simulink model "DATCOM_SimulinkModel"  (R2026a)
settings: Solver=ode4  StopTime=120  FixedStep=params.DT
InitFcn:
  | % Place this in SITL_SimulinkModel > Model Properties > Call Backs >
  | % InitFcn to initialize the states and stuff
  | fprintf("~~~~ Ardupilot SITL Time ~~~~~");
  | clear SITL_Link_Step
  | clear SITL_Bridge_Step
  | 
  | params = SITL_RascalParams();
  | paramsD = DATCOM_RascalParams();
  | params.DT = 1/1200;
  | 
  | %% Initial attitude
  | % Enter the required euler angles here
  | p = deg2rad(0);   % Phi - Roll angle
  | t = deg2rad(0);   % Theta - Pitch angle
  | s = deg2rad(0);   % Psi - Yaw angle
  | q = eul2quat([s t p]);
  | 
  | %% Initial velocity
  | % Glide test: 16 m/s along body x only, so AoA = 0
  | % (for level flight at a pitch angle use u = V*cos(t), w = V*sin(t))
  | u = 40;
  | w = 0;
  | 
  | %% Initial state
  | % Runway start (taildragger rest attitude)
  | % theta0 = deg2rad(14.3);
  | % X0 = [0;0;-0.4;  0;0;0;   cos(theta0/2);0;sin(theta0/2);0;  0;0;0];
  | X0 = [0;0;-2000;  16;0;0;  q';  0;0;0];    % 2000 m up so it doesn't hit the ground, north
  | 
  | %% Actuators and prop
  | PWM0 = 1500*ones(16,1);   % This is the systematic delay or else
  | % simulink thinks everything is happening at once!
  | delta0 = [0;0;0;0];       % For the aileron, elevator, rudder and throttle
  | % We are not considering a special one for the throttle as well
  | % This should also become the trim states if you are trying to
  | % start the SITL from a point in the Air
  | omega0 = 0;
  | 
  | %% Test PWM (throttle off). Elevator PWM sets the glide speed, 1500 = 0 rad
  | % above 1500 = nose up: dE = -(PWM-1500)/400*0.35 rad, e.g. 1569 -> -0.06
  | PWM_TEST = 1500*ones(16,1);
  | PWM_TEST(2) = 1580;
  | PWM_TEST(3) = 1100;
  | 
  | fprintf("~~~~ INITIALIZED ~~~~~");
StopFcn:
  | clear SITL_Link_Step
  | clear SITL_Bridge_Step
libraries: simulink_extras x3
settings Model: SimulationMode=accelerator  Creator=kiryuzerodev  LastModifiedBy=kiryuzerodev

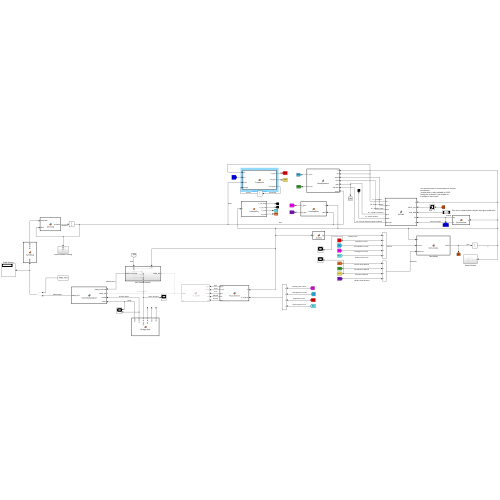
[thumbnail: Simulink's stored preview of the top-level diagram]
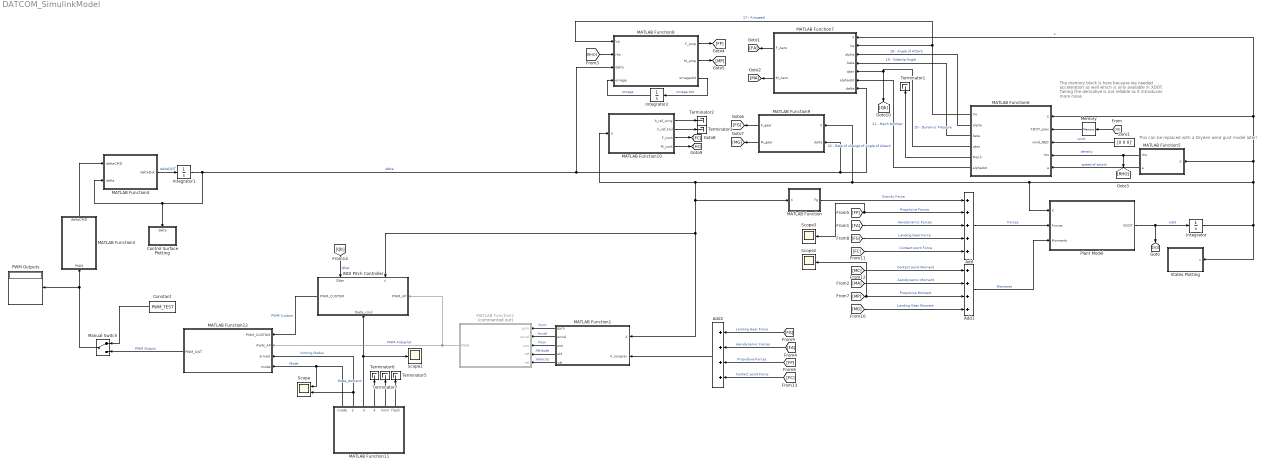
== system DATCOM_SimulinkModel ==
  note: The memory block is here because we needed acceleration
      |  as well which is only available in XDOT.
      | Taking the derivative is not reliable as
      | it introduces more noise
  note: This can be replaced with a Dryden wind gust model later!
  Add : Sum  Inputs=+++++
  Add1 : Sum  Inputs=++++
  Add2 : Sum  Inputs=++++
  Constant : Constant  Value=PWM_TEST
  Control Surface Plotting : Subsystem
  INDI Pitch Controller : Subsystem  TreatAsAtomicUnit=on
      settings: PortSchema="{\"entries\":[{\"content\":{\"sides\":[{\"content\":{\"connectorIds\":[\"In1\"]},\"type\":\"ConnectorPlacement.EquallySpacedRectSide\",\"uuid\":\"6d37aedf-8600-4591-b995-97b477a77a55\"},{\"content\":{\"connectorIds\":[\"Out1\"],\"side\":\"RIGHT\"},\"type\":\"ConnectorPlacement.EquallySpacedRectSide\",\"uuid\":\"78620349-e441-4417-9f68-6134c6dddec3\"},{\"content\":{\"connectorIds\":[\"In2\",\"In3\"],\"side\":\"TOP\"},\"type\":\"ConnectorPlacement.EquallySpacedRectSide\",\"uuid\":\"68daa815-3964-4591-9418-c320c8fdbef1\"},{\"content\":{\"connectorIds\":[\"In4\"],\"side\":\"BOTTOM\"},\"type\":\"ConnectorPlacement.EquallySpacedRectSide\",\"uuid\":\"2d52c1d4-1bc5-4ab7-be15-73a8ca1289f8\"}]},\"type\":\"ConnectorPlacement.EquallySpacedConnector\",\"uuid\":\"4e119030-0fd6-47a7-b3a8-f7366bb9867e\"}],\"packageUris\":[\"http://schema.mathworks.com/mf0/Connector/R2020b\"],\"version\":\"1.0\"}"
  Integrator : Integrator  InitialCondition=X0
  Integrator1 : Integrator  InitialCondition=delta0
  Integrator2 : Integrator  InitialCondition=omega0
  MATLAB Function : MATLAB Function  TreatAsAtomicUnit=on
  MATLAB Function1 : MATLAB Function  TreatAsAtomicUnit=on
  MATLAB Function10 : MATLAB Function  TreatAsAtomicUnit=on
  MATLAB Function11 : MATLAB Function  TreatAsAtomicUnit=on
  MATLAB Function12 : MATLAB Function  TreatAsAtomicUnit=on
  MATLAB Function2 : MATLAB Function  Commented=on  TreatAsAtomicUnit=on
  MATLAB Function3 : MATLAB Function  TreatAsAtomicUnit=on
  MATLAB Function4 : MATLAB Function  TreatAsAtomicUnit=on
  MATLAB Function5 : MATLAB Function  TreatAsAtomicUnit=on
  MATLAB Function6 : MATLAB Function  TreatAsAtomicUnit=on
  MATLAB Function7 : MATLAB Function  TreatAsAtomicUnit=on
  MATLAB Function8 : MATLAB Function  TreatAsAtomicUnit=on
  MATLAB Function9 : MATLAB Function  TreatAsAtomicUnit=on
  Manual Switch : ManualSwitch
  Memory : Memory  InitialCondition=zeros(13,1)
  PWM Outputs : Display
  Plant Model : MATLAB Function  TreatAsAtomicUnit=on
  Scope : Scope  NumInputPorts=2
  Scope1 : Scope
  Scope2 : Scope
      settings: ActiveDisplayYMinimum=-1  ActiveDisplayYMaximum=1  DataLoggingVariableName=ScopeData2
  Scope3 : Scope
      settings: ActiveDisplayYMinimum=-1  ActiveDisplayYMaximum=1  DataLoggingVariableName=ScopeData3
  States Plotting : Subsystem
  Terminator{1..3,5..7} (6 alike) : Terminator
  Zero1 : Constant  Value=[0 0 0]'  OutDataTypeStr=Inherit: Inherit via back propagation
  wires:
  Plant Model/1(XDOT) -> Integrator/1, [XD]  "xdot"
  Integrator/1 -> Plant Model/1(X), MATLAB Function9/1(X), MATLAB Function1/1(X), INDI Pitch Controller/2(x), MATLAB Function/1(X), MATLAB Function10/1(X), MATLAB Function7/1(X), MATLAB Function6/1(X), MATLAB Function5/1(X), States Plotting/1(x)  "x"
  MATLAB Function1/1(gyro) -> MATLAB Function2/1(gyro)  "Gyro"
  MATLAB Function1/2(accel) -> MATLAB Function2/2(accel)  "Accel"
  MATLAB Function1/3(pos) -> MATLAB Function2/3(pos)  "Posn"
  MATLAB Function1/4(att) -> MATLAB Function2/4(att)  "Attitude"
  MATLAB Function1/5(vel) -> MATLAB Function2/5(vel)  "Velocity"
  Add2/1 -> MATLAB Function1/2(F_nongrav)
  MATLAB Function4/1(deltaDot) -> Integrator1/1  "deltaDOT"
  Integrator1/1 -> MATLAB Function9/2(delta), MATLAB Function7/7(delta), MATLAB Function8/3(delta), MATLAB Function4/2(delta), Control Surface Plotting/1(delta)  "delta"
  MATLAB Function3/1(deltaCMD) -> MATLAB Function4/1(deltaCMD)
  MATLAB Function5/2(a) -> MATLAB Function6/5(a)  "speed of sound"
  MATLAB Function5/1(rho) -> [RHO], MATLAB Function6/4(rho)  "density"
  Memory/1 -> MATLAB Function6/2(XDOT_prev)
  [XD] -> Memory/1
  Zero1/1 -> MATLAB Function6/3(wind_NED)  "wind"
  MATLAB Function6/1(Va) -> MATLAB Function8/1(Va), MATLAB Function7/2(Va)  "17 - Airspeed"
  MATLAB Function6/2(alpha) -> MATLAB Function7/3(alpha)  "18 - Angle of Attack"
  MATLAB Function6/3(beta) -> MATLAB Function7/4(beta)  "19 - Sideslip Angle"
  MATLAB Function6/4(qbar) -> MATLAB Function7/5(qbar), [Qb]  "20 - Dynamic Pressure"
  MATLAB Function6/5(Mach) -> Terminator1/1  "21 - Mach Number"
  MATLAB Function6/6(alphadot) -> MATLAB Function7/6(alphadot)  "22 - Rate of change of Angle of Attack"
  MATLAB Function7/1(F_Aero) -> [FA]
  MATLAB Function7/2(M_Aero) -> [MA]
  [FA] -> Add/3  "Aerodynamic Forces"
  Add/1 -> Plant Model/2(Forces)  "Forces"
  Add1/1 -> Plant Model/3(Moments)  "Moments"
  [MA] -> Add1/2  "Aerodynamic Moment"
  [RHO] -> MATLAB Function8/2(rho)
  MATLAB Function/1(Fg) -> Add/1  "Gravity Force"
  [FA] -> Add2/2  "Aerodynamic Forces"
  MATLAB Function8/3(omegadot) -> Integrator2/1  "omega dot"
  Integrator2/1 -> MATLAB Function8/4(omega)  "omega"
  MATLAB Function8/1(F_prop) -> [FP]
  MATLAB Function8/2(M_prop) -> [MP]
  [FP] -> Scope3/1, Add/2  "Propulsive Forces"
  [FP] -> Add2/3  "Propulsive Forces"
  [MP] -> Scope2/1, Add1/3  "Propulsive Moment"
  MATLAB Function9/1(F_gear) -> [FG]
  MATLAB Function9/2(M_gear) -> [MG]
  [FG] -> Add/4  "Landing Gear Force"
  [FG] -> Add2/1  "Landing Gear Force"
  [MG] -> Add1/4  "Landing Gear Moment"
  Manual Switch/1 -> MATLAB Function3/1(PWM), PWM Outputs/1
  MATLAB Function10/1(h_ref_wing) -> Terminator2/1
  MATLAB Function10/2(h_ref_tail) -> Terminator3/1
  MATLAB Function10/3(F_cont) -> [FC]
  MATLAB Function10/4(M_cont) -> [MC]
  [FC] -> Add/5  "Contact point Force"
  [MC] -> Add1/1  "Contact point Moment"
  [FC] -> Add2/4  "Contact point Force"
  MATLAB Function11/3(theta_cmd) -> Scope1/1, INDI Pitch Controller/4(theta_cmd)  "theta_demand"
  Constant/1 -> Manual Switch/1
  INDI Pitch Controller/1(PWM_CUSTOM) -> MATLAB Function12/1(PWM_CUSTOM)  "PWM Custom"
  MATLAB Function11/2(armed) -> Scope/2, MATLAB Function12/3(armed)  "Arming Status"
  MATLAB Function11/1(mode) -> Scope/1, MATLAB Function12/4(mode)  "Mode"
  MATLAB Function2/1(PWM) -> INDI Pitch Controller/1(PWM_AP), MATLAB Function12/2(PWM_AP)  "PWM Ardupilot"
  MATLAB Function12/1(PWM_OUT) -> Manual Switch/2  "PWM Output"
  MATLAB Function11/4(phi_cmd) -> Terminator6/1
  MATLAB Function11/5(mnvr) -> Terminator7/1
  MATLAB Function11/6(fresh) -> Terminator5/1
  [Qb] -> INDI Pitch Controller/3(Qbar)  "Qbar"

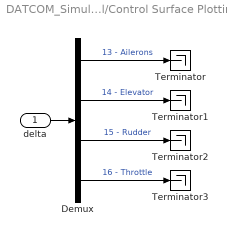
== system DATCOM_SimulinkModel/Control Surface Plotting ==
  delta : Inport
  Demux : Demux
  Terminator{,1..3} (4 alike) : Terminator
  wires:
  Demux/4 -> Terminator3/1  "16 - Throttle"
  Demux/1 -> Terminator/1  "13 - Ailerons"
  Demux/3 -> Terminator2/1  "15 - Rudder"
  Demux/2 -> Terminator1/1  "14 - Elevator"
  delta/1 -> Demux/1

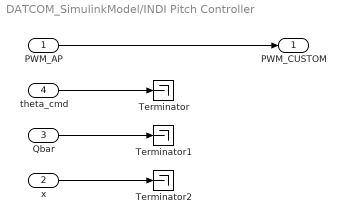
== system DATCOM_SimulinkModel/INDI Pitch Controller ==
  PWM_AP : Inport
  x : Inport  Port=2
  Qbar : Inport  Port=3
  theta_cmd : Inport  Port=4
  Terminator : Terminator
  Terminator1 : Terminator
  Terminator2 : Terminator
  PWM_CUSTOM : Outport
  wires:
  PWM_AP/1 -> PWM_CUSTOM/1
  theta_cmd/1 -> Terminator/1
  Qbar/1 -> Terminator1/1
  x/1 -> Terminator2/1

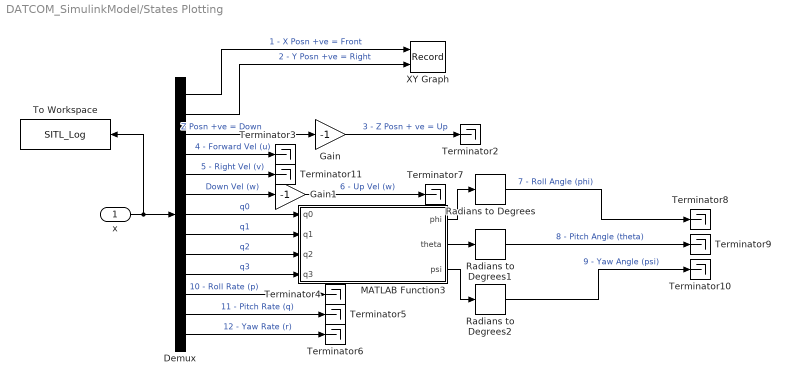
== system DATCOM_SimulinkModel/States Plotting ==
  x : Inport
  Demux : Demux  Outputs=13
  Gain : Gain  Gain=-1
  Gain1 : Gain  Gain=-1
  MATLAB Function3 : MATLAB Function  TreatAsAtomicUnit=on
  Radians to Degrees : simulink_extras/Transformations/Radians to Degrees
  Radians to Degrees1 : simulink_extras/Transformations/Radians to Degrees
  Radians to Degrees2 : simulink_extras/Transformations/Radians to Degrees
  Terminator{2..11} (10 alike) : Terminator
  To Workspace : ToWorkspace  VariableName=SITL_Log  SampleTime=-1
  XY Graph : Record  NumPorts=2.0  FileSettingsInternal="{\"entries\":[{\"content\":{\"excelSettings\":{\"content\":{},\"type\":\"Streamout.ExcelSettings\"},\"parquetSettings\":{\"content\":{},\"type\":\"Streamout.ParquetSettings\"}},\"type\":\"Streamout.FileSettingStorage\",\"uuid\":\"\"}],\"packageUris\":[\"http:\\/\\/schema.mathworks.com\\/mf0\\/streamout_blocks\\/R2020a\"],\"version\":\"1.0\"}"  FrameSettings=[0, 0]  Layout=[1 1]  SignalsInternal="{\"entries\":[{\"content\":{\"signals\":[{\"content\":{\"blockPath\":[],\"dimensions\":[1,1],\"domain\":\"\",\"lineColor\":\"#77ac30\",\"lineWidth\":2,\"plots\":[ 1 ],\"port\":1,\"sid\":[\"\"],\"signalID\":1,\"signalName\":\"1 - X Posn +ve = Front\"},\"type\":\"RecordBlkView.Signal\",\"uuid\":\"\"},{\"content\":{\"blockPath\":[],\"dimensions\":[1,1],\"domain\":\"\",\"lineColor\":\"#4dbeee\",\"lineWidth\":2,\"plots\":[ 1 ],\"port\":2,\"sid\":[\"\"],\"signalID\":2,\"signalName\":\"2 - Y Posn +ve = Right\"},\"type\":\"RecordBlkView.Signal\",\"uuid\":\"\"}]},\"type\":\"RecordBlkView.InputSignals\",\"uuid\":\"\"}],\"packageUris\":[\"http:\\/\\/schema.mathworks.com\\/mf0\\/streamout_blocks\\/R2020a\"],\"version\":\"1.0\"}"  VisualizationBindings="{\"xyplotplugin\":{\"info\":[{\"series\":[{\"bindingParametersList\":[{\"parameter\":\"X-Axis\",\"signalID\":1,\"signalName\":\"1 - X Posn +ve = Front\"},{\"parameter\":\"Y-Axis\",\"signalID\":2,\"signalName\":\"2 - Y Posn +ve = Right\"}],\"seriesID\":0}],\"subplotID\":1}]}}"  CompatibilityTag=XY
  wires:
  MATLAB Function3/2(theta) -> Radians to Degrees1/1
  Demux/1 -> XY Graph/1  "1 - X Posn +ve = Front"
  Demux/9 -> MATLAB Function3/3(q2)  "q2"
  Demux/4 -> Terminator3/1  "4 - Forward Vel (u)"
  Demux/5 -> Terminator11/1  "5 - Right Vel (v)"
  Demux/6 -> Gain1/1  "Down Vel (w)"
  Demux/3 -> Gain/1  "Z Posn +ve = Down"
  Demux/13 -> Terminator6/1  "12 - Yaw Rate (r)"
  Demux/7 -> MATLAB Function3/1(q0)  "q0"
  Demux/2 -> XY Graph/2  "2 - Y Posn +ve = Right"
  Demux/8 -> MATLAB Function3/2(q1)  "q1"
  Demux/12 -> Terminator5/1  "11 - Pitch Rate (q)"
  Demux/10 -> MATLAB Function3/4(q3)  "q3"
  MATLAB Function3/3(psi) -> Radians to Degrees2/1
  Demux/11 -> Terminator4/1  "10 - Roll Rate (p)"
  MATLAB Function3/1(phi) -> Radians to Degrees/1
  Gain/1 -> Terminator2/1  "3 - Z Posn + ve = Up"
  Gain1/1 -> Terminator7/1  "6 - Up Vel (w)"
  x/1 -> To Workspace/1, Demux/1
  Radians to Degrees/1 -> Terminator8/1  "7 - Roll Angle (phi)"
  Radians to Degrees1/1 -> Terminator9/1  "8 - Pitch Angle (theta)"
  Radians to Degrees2/1 -> Terminator10/1  "9 - Yaw Angle (psi)"

== matlab function DATCOM_SimulinkModel/MATLAB Function7 ==
  data: X input; Va input; alpha input; beta input; qbar input; alphadot input; paramsD parameter; F_Aero output; delta input; M_Aero output
function [F_Aero,M_Aero] = Aerodynamics(X,Va, alpha, beta, qbar, alphadot, paramsD,delta)
[F_Aero,M_Aero] = DATCOM_Aerodynamics(X, Va, alpha, beta, qbar, alphadot, paramsD,delta);

== matlab function DATCOM_SimulinkModel/MATLAB Function8 ==
  data: Va input; rho input; delta input; omega input; F_prop output; M_prop output; omegadot output; paramsD parameter
function [F_prop, M_prop, omegadot] = Propulsion(Va, rho, delta,omega,paramsD)
[F_prop, M_prop, omegadot] = SITL_Propulsion(Va, rho, delta,omega,paramsD);

== matlab function DATCOM_SimulinkModel/MATLAB Function9 ==
  data: X input; F_gear output; delta input; M_gear output; params parameter
function [F_gear,M_gear]=LandingGear(X,delta,params)
[F_gear,M_gear]=SITL_LandingGear(X,delta,params);

== matlab function DATCOM_SimulinkModel/MATLAB Function10 ==
  data: X input; h_ref_wing output; h_ref_tail output; F_cont output; M_cont output; paramsD parameter
function [h_ref_wing, h_ref_tail, F_cont, M_cont] = ContactPhy(X, paramsD)
[h_ref_wing, h_ref_tail, F_cont, M_cont] = SITL_ContactPhysiscs(X, paramsD);

== matlab function DATCOM_SimulinkModel/MATLAB Function11 ==
  settings: updateMethod=DISCRETE  sampleTime=0.02
  data: mode output; armed output; theta_cmd output; phi_cmd output; mnvr output; fresh output
function [mode,armed,theta_cmd, phi_cmd,  mnvr, fresh] = Bridge_Step()
coder.extrinsic('SITL_Bridge_Step');
theta_cmd = 0; phi_cmd = 0; armed = 0; mode = 0; mnvr = 0; fresh = 0;
[theta_cmd, phi_cmd, armed, mode, mnvr, fresh] = SITL_Bridge_Step();
% This has to have sample time = 0.02s as it is the link between MAVLink
% and MATLAB

== matlab function DATCOM_SimulinkModel/MATLAB Function ==
  data: X input; Fg output; paramsD parameter
function Fg = Gravity(X, paramsD)
Fg = SITL_Gravity(X, paramsD);

== matlab function DATCOM_SimulinkModel/MATLAB Function12 ==
  data: PWM_CUSTOM input size=[16 1]; PWM_AP input size=[16 1]; PWM_OUT output; armed input size=[1 1]; mode input; paramsD parameter
function PWM_OUT = ControllerSelection(PWM_CUSTOM,PWM_AP, armed, mode, paramsD)
PWM_OUT = SITL_ControlSelect(PWM_AP, PWM_CUSTOM, armed, mode, paramsD);

== matlab function DATCOM_SimulinkModel/Plant Model ==
  data: X input size=13; XDOT output; Forces input; Moments input; paramsD parameter
function XDOT = DoF_6_Eqns(X, Forces, Moments, paramsD)
XDOT = zeros(13,1);
XDOT = SITL_6DoFEqns(X, Forces, Moments, paramsD);

== matlab function DATCOM_SimulinkModel/MATLAB Function1 ==
  data: X input; gyro output; F_nongrav input; accel output; pos output; att output; vel output; paramsD parameter
function [gyro, accel, pos, att, vel] = True_Sensors(X, F_nongrav, paramsD)
[gyro, accel, pos, att, vel] = SITL_Sensors(X, F_nongrav, paramsD);

== matlab function DATCOM_SimulinkModel/MATLAB Function2 ==
  settings: updateMethod=DISCRETE  sampleTime=params.DT
  data: gyro input; PWM output; accel input; pos input; att input; vel input
function PWM = SITL_Linker(gyro, accel, pos, att, vel)
coder.extrinsic('SITL_Link_Step');   % run this one in normal MATLAB
PWM = zeros(16,1);                   % tell Simulink the output size
PWM = SITL_Link_Step(gyro, accel, pos, att, vel);
% This function cannot run more times in 1 second which was happening when
% solving. Set it to run exactly the number of times as the simulation per
% step

== matlab function DATCOM_SimulinkModel/States Plotting/MATLAB Function3 ==
  data: phi output; theta output; psi output; q0 input; q1 input; q2 input; q3 input
function [phi,theta,psi] = Quat2Euler(q0,q1,q2,q3)
[phi,theta,psi] = SITL_Quat2Euler(q0,q1,q2,q3);

== matlab function DATCOM_SimulinkModel/MATLAB Function3 ==
  data: deltaCMD output; PWM input size=[16 1]; paramsD parameter
function deltaCMD = ServoMap(PWM,paramsD)
deltaCMD = SITL_ServoMap(PWM,paramsD);

== matlab function DATCOM_SimulinkModel/MATLAB Function4 ==
  data: deltaDot output; deltaCMD input; delta input; paramsD parameter
function deltaDot = ServoLag(deltaCMD,delta,paramsD)
deltaDot = SITL_ServoLag(deltaCMD,delta,paramsD);

== matlab function DATCOM_SimulinkModel/MATLAB Function5 ==
  data: X input; rho output; a output; paramsD parameter
function [rho, a] = Environment(X, paramsD)
[rho, a] = SITL_Environment(X, paramsD);

== matlab function DATCOM_SimulinkModel/MATLAB Function6 ==
  data: X input; Va output; XDOT_prev input; wind_NED input; rho input; a input; alpha output; beta output; qbar output; Mach output; alphadot output
function [Va, alpha, beta, qbar, Mach,  alphadot] = AirData(X, XDOT_prev, wind_NED, rho, a)
[Va, alpha, beta, qbar, Mach, alphadot] = SITL_AirData(X, XDOT_prev, wind_NED, rho, a);
